simulink model "PWM_Sampling"  (R2024b)
settings: Solver=ode15s  StartTime=0.0  StopTime=0.04  RelTol=1e-3  AbsTol=1e-3  EnableMultiTasking=on
libraries: fl_lib x6, nesl_utility x4, ee_lib x3
CloseFcn:
  | try,close(h1_ee_motor_dc_pwm),end
  | clear h1_ee_motor_dc_pwm
  | 
  | clear simlog_ee_motor_dc_pwm
  | clear logsout_ee_motor_dc_pwm
  | clear RPM RPM1 tout
Description:
  | PWM-Controlled DC Motor
settings Model: Creator=The MathWorks, Inc.  LastModifiedBy=student
settings SolverCC: AutoScaleAbsTol=off  AlgebraicLoopSolver=TrustRegion
settings DataIOCC: LimitDataPoints=on  MaxDataPoints=10000  SaveFormat=Array  ReturnWorkspaceOutputs=off  SignalLoggingName=logsout_ee_motor_dc_pwm
settings OptimizationCC: ExpressionDepthLimit=2147483647  InitFltsAndDblsToZero=on  LifeSpan=inf
settings DebuggingCC: UnderspecifiedInitializationDetection=Classic  MergeDetectMultiDrivingBlocksExec=none  FcnCallInpInsideContextMsg=warning  UnconnectedInputMsg=warning  UnconnectedOutputMsg=warning  UnconnectedLineMsg=warning  StateNameClashWarn=warning  SFUnexpectedBacktrackingDiag=warning  SFNoUnconditionalDefaultTransitionDiag=warning  SFExecutionAtInitializationDiag=none  ArithmeticOperatorsInVariantConditions=warning
settings HardwareCC: ProdBitPerPointer=32  ProdBitPerSizeT=32  ProdBitPerPtrDiffT=32  ProdLargestAtomicFloat=None  ProdIntDivRoundTo=Undefined  ProdEndianess=Unspecified  ProdWordSize=32  ProdHWDeviceType=32-bit Generic
settings ModelReferenceCC: EnableRefExpFcnMdlSchedulingChecks=on  PropagateSignalLabelsOutOfModel=off
settings SFSimCC: SimUseLocalCustomCode=off  CustomCodeUndefinedFunction=UseInterfaceOnly
settings RTWCC: RTWUseLocalCustomCode=off  GPUComputeCapability=3.5  DLArmComputeVersion=19.05
settings CodeAppCC: StateflowObjectComments=on
settings GRTTargetCC: TargetLangStandard=C89/C90 (ANSI)  CombineOutputUpdateFcns=off  GRTInterface=on
settings ConfigComp: CovMetricSettings=dw  CovSaveCumulativeToWorkspaceVar=on  CovSaveSingleToWorkspaceVar=on  CovExternalEMLEnable=off  CovSFcnEnable=off
settings SimscapeCC: SimscapeLogType=all  SimscapeLogSimulationStatistics=on  SimscapeLogName=simlog_ee_motor_dc_pwm  SimscapeLogDataHistory=10000

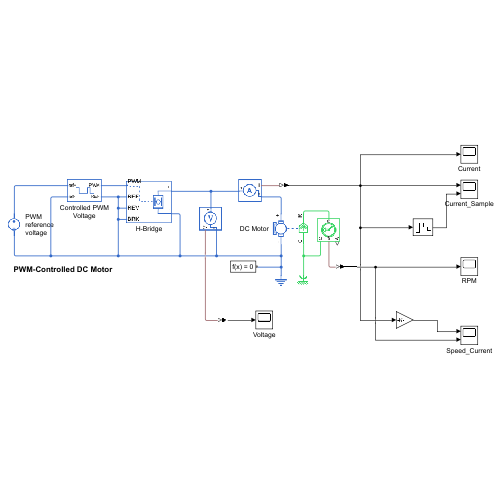
[thumbnail: Simulink's stored preview of the top-level diagram]
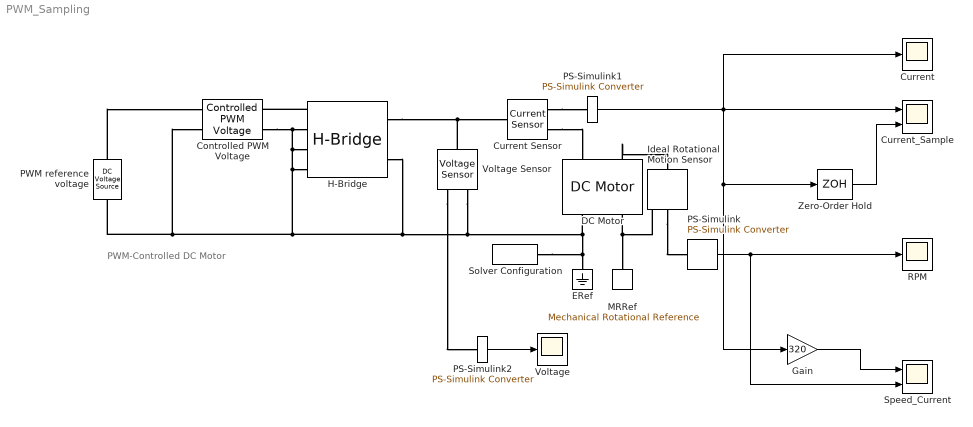
== system PWM_Sampling ==
  note: PWM-Controlled DC Motor
  Controlled PWM Voltage : ee_lib/Integrated Circuits/Controlled PWM Voltage  F=10000 Hz  TD=0.000025 s  pulse_width_offset=0 s  pulse_min=0 s  pwm_or_av=ee.enum.pwm_or_av.pwm  event_type=1  sample_time=5e-6 s  Vmin=0 V  Vmax=5 V  Vm=5 V  u_min=0  u_max=1
  Current : Scope
  Current Sensor : fl_lib/Electrical/Electrical Sensors/Current Sensor
  Current_Sample : Scope  NumInputPorts=2
  DC Motor : ee_lib/Electromechanical/Brushed Motors/DC Motor  field_option=ee.enum.field_option.pm  Rf=100 Ohm  Lf=1 H  Laf=0.15 H  If0=0 A  parameterization=ee.enum.dcparam_option.circuit_param  Ra=3.2 Ohm  La=0.0041 H  emf_or_torque=ee.enum.emf_or_torque.kv  Kv=0.12 V/(rad/s)  Ki=6.876e-04 N*m/A  T_stall=0.1 N*m  w_max=4000 rpm  w_rated=2500 rpm  P_rated=10 W  V_rated=12 V  lam_param=ee.enum.lam_param.current  i_noload=0.3 A  V_i_noload=24 V  J=3.52e-5 kg*m^2  lam=0.5e-5 N*m/(rad/s)  speed0=0 rpm  t_fault_armature=1 s  t_fault_field=1 s  fault_action=simscape.enum.assert.action.none  alpha=3.93e-3 1/K  Tmeas=25 degC  thermal_mass=100 J/K  initial_temperature=25 degC
  ERef : fl_lib/Electrical/Electrical Elements/Electrical Reference
  Gain : Gain  Gain=320
  H-Bridge : ee_lib/Semiconductors & Converters/Converters/H-Bridge  supply_ports=ee.enum.supply_ports.hidesupply  pwm_or_av=ee.enum.pwm_or_av.averaged  regenerative_braking_mode=ee.enum.converters.regenerative_braking_mode.always_enabled  discontinuous=ee.enum.current_profile.continuous  freewheeling_mode=ee.enum.converters.freewheeling_mode.one_switch_one_diode  Rload=3.38+0.1 Ohm  Lload=1e-5 H  F=4 kHz  Venable=2.5 V  Vmax=5 V  Vreverse=2.5 V  Vbrake=2.5 V  Vm=12 V  Ron=0.1 Ohm  Don=0.1 Ohm  Goff=1e-6 S  Tmeas=298.15 K  Ron2=0.1 Ohm  Don2=0.05 Ohm  Tmeas2=398.15 K  thermal_mass=100 J/K  initial_temperature=298.15 K
  Ideal Rotational Motion Sensor : fl_lib/Mechanical/Mechanical Sensors/Ideal Rotational Motion Sensor  reference=foundation.enum.MeasurementReference.difference  acceleration_port=false  velocity_port=true  position_port=true  wrap_angle=simscape.enum.onoff.off  offset=0 deg
  MRRef : fl_lib/Mechanical/Rotational Elements/Mechanical Rotational Reference
  PS-Simulink : nesl_utility/PS-Simulink Converter  PhysicalDomain=network_engine_domain  SubClassName=ps_output  LeftPortType=input  RightPortType=output  PseudoPeriodic=off  Frequencies=[]  VectorFormat=1-D array  Unit=rpm  AffineConversion=off
  PS-Simulink1 : nesl_utility/PS-Simulink Converter  PhysicalDomain=network_engine_domain  SubClassName=ps_output  LeftPortType=input  RightPortType=output  PseudoPeriodic=off  Frequencies=[]  VectorFormat=1-D array  Unit=A  AffineConversion=off
  PS-Simulink2 : nesl_utility/PS-Simulink Converter  PhysicalDomain=network_engine_domain  SubClassName=ps_output  LeftPortType=input  RightPortType=output  PseudoPeriodic=off  Frequencies=[]  VectorFormat=1-D array  Unit=V  AffineConversion=off
  PWM reference voltage : fl_lib/Electrical/Electrical Sources/DC Voltage Source  v0=2.5 V
  RPM : Scope
  Solver Configuration : nesl_utility/Solver Configuration  PhysicalDomain=network_engine_domain  SubClassName=solver  LeftPortType=input  RightPortType=generic  Tones=[]  Harmonics=[]  SimulateNoise=off  Profile=off  UseLocalSampling=off  EnableSwitchedLinearOptims=on  FrequencyDomain=off  UseCCode=off  RelTol=0.001  AbsTol=1e-06  MinStep=1e-09  ToWorkspace=off  RevertToSquareIcSolve=off  NumHomotopyIterations=100  PhasorMode=off  PhasorModeNumHarmonics=1  ConsistencySolver=NEWTON_FTOL  IndexReductionMethod=DerivativeReplacement  DoDC=off  ResidualTolerance=1e-9  ConsistencyTolSource=GLOBAL  ConsistencyAbsTol=0.001  ConsistencyRelTol=0.001  ConsistencyTolFactor=0.001  UseLocalSolver=off  LocalSolverChoice=NE_BACKWARD_EULER_ADVANCER  ResolveIndetEquations=on  FunctionEvalNumThread=1  LocalSolverSampleTime=5e-6  DoFixedCost=off  MaxNonlinIter=4  MaxModeIter=2  ComputeImpulses=off  ImpulseIterations=2  LinearAlgebra=auto  LinearAlgebraNumThread=0  EquationFormulation=NE_TIME_EF  DelaysMemoryBudget=1024  AutomaticFiltering=on  FilteringTimeConstant=0.001  PartitionStorageMethod=AS_NEEDED  PartitionMemoryBudget=1024  PartitionMethod=FAST  MultibodyUseLocalSolver=off  MultibodyLocalSolverChoice=ODE1  MultibodyLocalSolverSampleTime=0.001
  Speed_Current : Scope  NumInputPorts=2
  Voltage : Scope
  Voltage Sensor : fl_lib/Electrical/Electrical Sensors/Voltage Sensor
  Zero-Order Hold : ZeroOrderHold  SampleTime=0.0001
  wires:
  PS-Simulink/1 -> RPM/1, Speed_Current/2
  PS-Simulink1/1 -> Current/1, Current_Sample/1, Zero-Order Hold/1, Gain/1
  Zero-Order Hold/1 -> Current_Sample/2
  Gain/1 -> Speed_Current/1
  PS-Simulink2/1 -> Voltage/1
  connections:
  DC Motor/LConn2 -- Ideal Rotational Motion Sensor/LConn1
  H-Bridge/LConn1 -- Controlled PWM Voltage/RConn1
  DC Motor/RConn2 -- MRRef/LConn1 -- Ideal Rotational Motion Sensor/RConn1
  Ideal Rotational Motion Sensor/RConn2 -- PS-Simulink/LConn1
  PWM reference voltage/LConn1 -- Controlled PWM Voltage/LConn1
  H-Bridge/RConn1 -- Voltage Sensor/LConn1 -- Current Sensor/LConn1
  Current Sensor/RConn2 -- DC Motor/LConn1
  Current Sensor/RConn1 -- PS-Simulink1/LConn1
  Voltage Sensor/RConn2 -- DC Motor/RConn1 -- Solver Configuration/RConn1 -- ERef/LConn1 -- H-Bridge/RConn2 -- PWM reference voltage/RConn1 -- Controlled PWM Voltage/LConn2 -- H-Bridge/LConn2 -- Controlled PWM Voltage/RConn2 -- H-Bridge/LConn3 -- H-Bridge/LConn4
  Voltage Sensor/RConn1 -- PS-Simulink2/LConn1
